simulink model "simula_distancia2026"  (R2024b)
settings: Solver=FixedStepAuto  StartTime=0.0  StopTime=tfin  FixedStep=ts  RelTol=1e-6  AbsTol=1e-6
values from neighbouring files (symbols this model uses):
  b = 0.75    [Ensayo 9_2.mat]    (also in EnsayoRobot.m = 1; Ensayo_7_3.mat = 1; Ensayo_8_3.mat; Ini_simulador2026.m)
  D = 0.15772    [Ensayo 9_2.mat]    (also in Ensayo1.mat = 0.074118; Ensayo10.mat = 0.074118; Ensayo11.mat = 0.074118; Ensayo2.mat = 0.074118)
  d1 = 0    [Ensayo 9_2.mat]    (also in Ensayo_7_3.mat; Ensayo_8_3.mat; Ini_simulador2026.m)
  flag_curva = 1    [Ensayo 9_2.mat]    (also in Ensayo_7_3.mat; Ensayo_8_3.mat; Ini_simulador2026.m)
  K1 = 0.028057    [Ensayo 9_2.mat]    (also in Ensayo_7_3.mat; Ensayo_8_3.mat; Ini_simulador2026.m)
  Kext = 18    [Ensayo 9_2.mat]    (also in Ensayo_7_3.mat = 25; Ensayo_8_3.mat; Ini_simulador2026.m; parameters_8.m)
  Kint = 80    [Ensayo 9_2.mat]    (also in Ensayo_7_3.mat; Ensayo_8_3.mat; Ini_simulador2026.m)
  Km = 0.0020745    [Ensayo 9_2.mat]    (also in Ensayo1.mat; Ensayo10.mat; Ensayo11.mat; Ensayo2.mat)
  N = 8    [Ensayo 9_2.mat]    (also in EnsayoRobot.m = 3; Ensayo_7_3.mat; Ensayo_8_3.mat; Ini_simulador2026.m)
  periodo = 37    [Ensayo 9_2.mat]    (also in Ensayo_7_3.mat = 60; Ensayo_8_3.mat = 60; Ini_simulador2026.m = floor(periodo*0.1/Ref_Vo))
  Ref_Vo = 0.16    [Ensayo 9_2.mat]    (also in Ensayo_7_3.mat = 0.1; Ensayo_8_3.mat = 0.1; Ini_simulador2026.m)
  T1 = 0    [Ensayo 9_2.mat]    (also in Ensayo_7_3.mat; Ensayo_8_3.mat; Ini_simulador2026.m)
  t_fin_curva = 18.3904862255    [Ensayo 9_2.mat]    (also in Ensayo_7_3.mat = 29.4247779608; Ensayo_8_3.mat = 29.4247779608; Ini_simulador2026.m)
  t_ini_curva = 12.5    [Ensayo 9_2.mat]    (also in Ensayo_7_3.mat = 20; Ensayo_8_3.mat = 20; Ini_simulador2026.m)
  Td = 0    [Ensayo 9_2.mat]    (also in EnsayoRobot.m = 0.012; Ensayo_7_3.mat; Ensayo_8_3.mat; Ini_simulador2026.m)
  Ti = 5    [Ensayo 9_2.mat]    (also in Ensayo1.mat = 0.06; Ensayo10.mat = 0.02; Ensayo11.mat = 0.02; Ensayo2.mat = 0.06)
  tiempo_step_d = 6    [Ensayo 9_2.mat]    (also in Ensayo_7_3.mat = 10; Ensayo_8_3.mat = 10; Ini_simulador2026.m = floor(tiempo_step_d*0.1/Ref_Vo))
  Vo = 0.16    [Ensayo 9_2.mat]    (also in Ensayo_7_3.mat = 0.1; Ensayo_8_3.mat = 0.1; Ini_simulador2026.m)
settings Model: Creator=ramonimac  LastModifiedBy=laboratorios
settings DataIOCC: ReturnWorkspaceOutputs=off
settings RTWCC: GPUComputeCapability=3.5

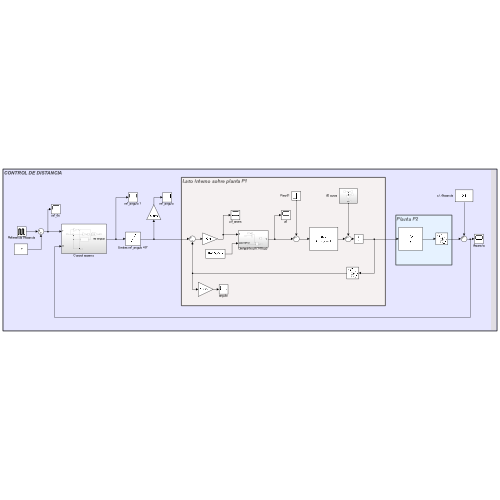
[thumbnail: Simulink's stored preview of the top-level diagram]
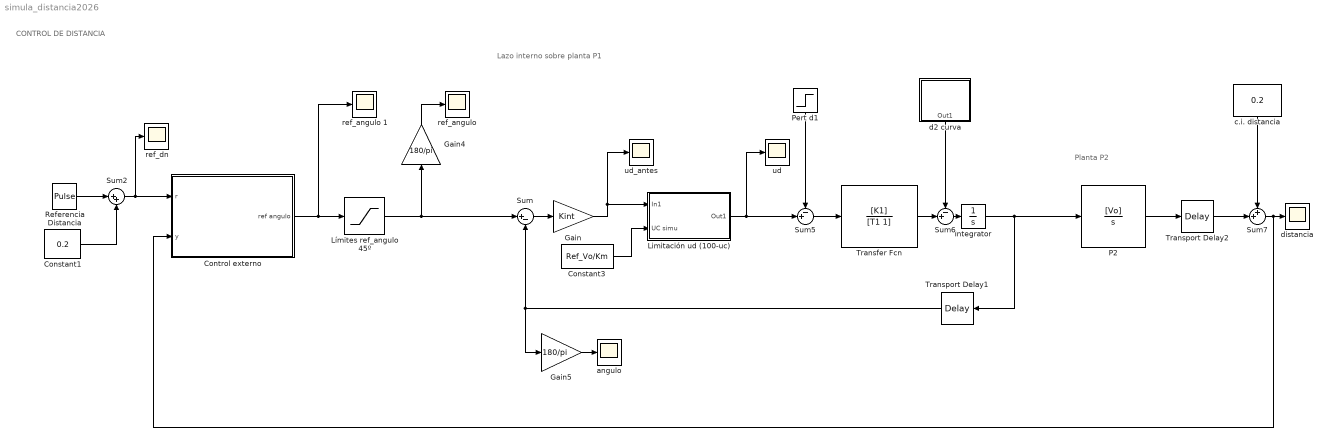
== system simula_distancia2026 ==
  note: Planta P2
  note: CONTROL DE DISTANCIA
  note: Lazo interno sobre planta P1
  Constant1 : Constant  Value=0.2
  Constant3 : Constant  Value=Ref_Vo/Km
  Control externo : Subsystem
  Gain : Gain  Gain=Kint
  Gain4 : Gain  Gain=180/pi
  Gain5 : Gain  Gain=180/pi
  Integrator : Integrator
  Limitación ud (100-uc) : Subsystem
  Límites ref_angulo 45º : Saturate  UpperLimit=pi/4  LowerLimit=-pi/4
  P2 : TransferFcn  Numerator=[Vo]  Denominator=[1 0]
  Pert d1 : Step  Time=20  After=d1  SampleTime=0
  Referencia Distancia : DiscretePulseGenerator  PulseType=Time based  Amplitude=single(0.02)  Period=periodo  PulseWidth=50  PhaseDelay=tiempo_step_d  SampleTime=500
  Sum : Sum  Inputs=|+-
  Sum2 : Sum  Inputs=|++
  Sum5 : Sum  Inputs=-+|
  Sum6 : Sum  Inputs=-+|
  Sum7 : Sum  Inputs=++|
  Transfer Fcn : TransferFcn  Numerator=[K1]  Denominator=[T1 1]
  Transport Delay1 : TransportDelay  DelayTime=D
  Transport Delay2 : TransportDelay  DelayTime=D
  angulo : Scope
  c.i. distancia : Constant  Value=0.2
  d2 curva : Subsystem
  distancia : Scope
  "ref_angulo " : Scope
  ref_angulo 1 : Scope
  ref_dn : Scope
  ud : Scope
  ud_antes : Scope
  wires:
  Sum/1 -> Gain/1
  Sum2/1 -> ref_dn/1, Control externo/1(r)
  Referencia Distancia/1 -> Sum2/1
  Constant1/1 -> Sum2/2
  Gain4/1 -> "ref_angulo "/1
  Sum5/1 -> Transfer Fcn/1
  Gain5/1 -> angulo/1
  Pert d1/1 -> Sum5/1
  Transfer Fcn/1 -> Sum6/2
  Sum6/1 -> Integrator/1
  Transport Delay1/1 -> Gain5/1, Sum/2
  Limitación ud (100-uc)/1(Out1) -> ud/1, Sum5/2
  Límites ref_angulo 45º/1 -> Sum/1, Gain4/1
  Constant3/1 -> Limitación ud (100-uc)/2(UC simu)
  P2/1 -> Transport Delay2/1
  Integrator/1 -> P2/1, Transport Delay1/1
  d2 curva/1(Out1) -> Sum6/1
  Gain/1 -> Limitación ud (100-uc)/1(In1), ud_antes/1
  Sum7/1 -> Control externo/2(y), distancia/1
  Transport Delay2/1 -> Sum7/2
  c.i. distancia/1 -> Sum7/1
  Control externo/1(ref angulo) -> Límites ref_angulo 45º/1, ref_angulo 1/1

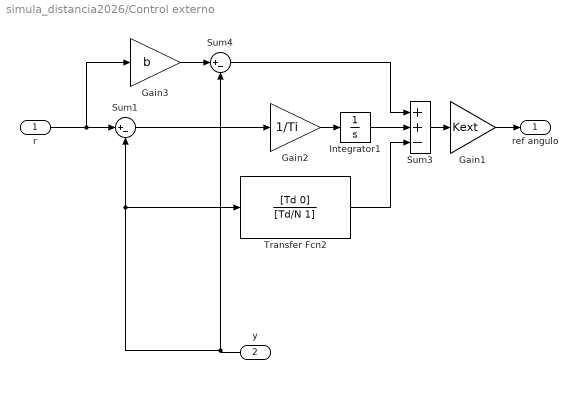
== system simula_distancia2026/Control externo ==
  r : Inport
  y : Inport  Port=2
  Gain1 : Gain  Gain=Kext
  Gain2 : Gain  Gain=1/Ti
  Gain3 : Gain  Gain=b
  Integrator1 : Integrator  InitialCondition=0.2*(1-b)*1
  Sum1 : Sum  Inputs=|+-
  Sum3 : Sum  Inputs=++-
  Sum4 : Sum  Inputs=|+-
  Transfer Fcn2 : TransferFcn  Numerator=[Td 0]  Denominator=[Td/N 1]
  ref angulo : Outport
  wires:
  Sum1/1 -> Gain2/1
  y/1 -> Sum4/2, Transfer Fcn2/1, Sum1/2
  Transfer Fcn2/1 -> Sum3/3
  Gain3/1 -> Sum4/1
  Gain1/1 -> ref angulo/1
  Integrator1/1 -> Sum3/2
  Sum3/1 -> Gain1/1
  Gain2/1 -> Integrator1/1
  Sum4/1 -> Sum3/1
  r/1 -> Gain3/1, Sum1/1

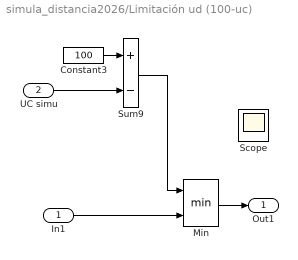
== system simula_distancia2026/Limitación ud (100-uc) ==
  In1 : Inport
  UC simu : Inport  Port=2
  Constant3 : Constant  Value=100
  Min : MinMax  Inputs=2
  Scope : Scope
  Sum9 : Sum  Inputs=+-
  Out1 : Outport
  wires:
  Min/1 -> Out1/1
  In1/1 -> Min/2
  Sum9/1 -> Min/1
  Constant3/1 -> Sum9/1
  UC simu/1 -> Sum9/2

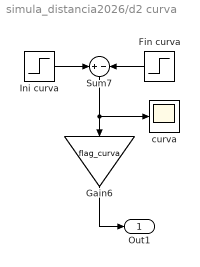
== system simula_distancia2026/d2 curva ==
  Fin curva : Step  Time=t_fin_curva  After=pi/(t_fin_curva-t_ini_curva)  SampleTime=0
  Gain6 : Gain  Gain=flag_curva
  Ini curva : Step  Time=t_ini_curva  After=pi/(t_fin_curva-t_ini_curva)  SampleTime=0
  Sum7 : Sum  Inputs=+|-
  curva : Scope
  Out1 : Outport
  wires:
  Sum7/1 -> curva/1, Gain6/1
  Fin curva/1 -> Sum7/2
  Gain6/1 -> Out1/1
  Ini curva/1 -> Sum7/1
